simulink model "hopper_3dof_cascade_2"  (R2025a)
settings: Solver=VariableStepAuto  StartTime=0.0  StopTime=36  MaxStep=.005  RelTol=1e-3
values from neighbouring files (symbols this model uses):
  AVI = size_avionics(IN)    [main.m]
  bp = data(:,1)    [load_lookup.m]
  ENGINE = size_engine(IN)    [main.m]
  IN = mission_inputs()    [main.m]
  OUT = Outputs(IN, VEH, TANKS, STRUCT)    [main.m]
  TANKS = size_tanks(IN)    [main.m]
  tbl1 = data(:,2)    [load_lookup.m]
  tbl2 = data(:,3)    [load_lookup.m]
libraries: slpidlib x6, SignalEditorBlockLib x1, cstblocks x1, dspsrcs4 x1
(part 1 of 2)
settings Model: Creator=Espin  LastModifiedBy=asing
settings DebuggingCC: AlgebraicLoopMsg=none

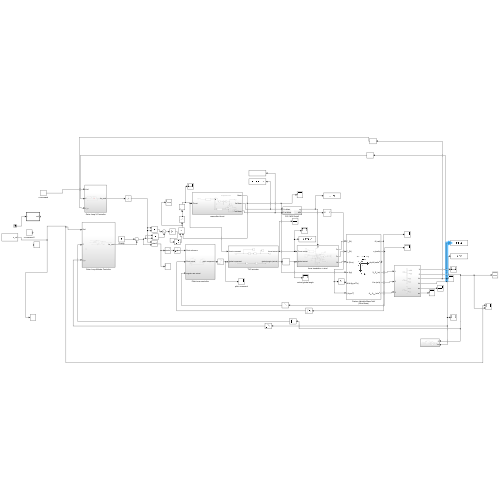
[thumbnail: Simulink's stored preview of the top-level diagram]
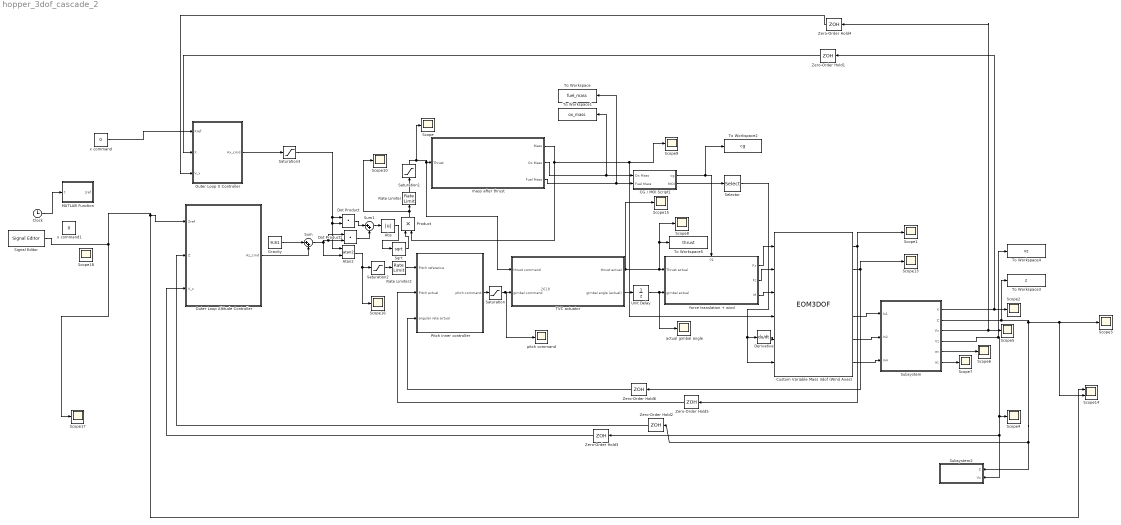
== system hopper_3dof_cascade_2 ==
  note: .2618
  Abs : Abs  SaturateOnIntegerOverflow=off
  Atan2 : Trigonometry  Operator=atan2
  CG / MOI Script1 : Subsystem
  Clock : Clock
  Custom Variable Mass 3dof (Wind Axes) : EOM3DOF  mtype=Custom Variable  v_ini=0
  Derivative : Derivative
  Dot Product : DotProduct  OutDataTypeStr=Inherit: Inherit via internal rule
  Dot Product1 : DotProduct  OutDataTypeStr=Inherit: Inherit via internal rule
  Gravity : Constant  Value=9.81
  MATLAB Function : MATLAB Function  TreatAsAtomicUnit=on
  Outer Loop Altitude Controller : Subsystem
  Outer Loop X Controller : Subsystem
  Pitch inner controller : Subsystem
  Product : Product
  Rate Limiter : RateLimiter  RisingSlewLimit=800  FallingSlewLimit=-800  SampleTimeMode=inherited
  Rate Limiter2 : RateLimiter  RisingSlewLimit=.2618  FallingSlewLimit=-.2618  SampleTimeMode=inherited
  Saturation : Saturate  UpperLimit=.25  LowerLimit=-.25
  Saturation1 : Saturate  UpperLimit=2400  LowerLimit=890  ZeroCross=off
  Saturation2 : Saturate  UpperLimit=.1  LowerLimit=-.1
  Saturation3 : Saturate  UpperLimit=.8  LowerLimit=-.8
  Scope{,1..10,13,15..18} (16 alike) : Scope
      Scope settings: ActiveDisplayYMinimum=624.4996725299402  ActiveDisplayYMaximum=2705.46842252994  DataLoggingVariableName=ScopeData17
      Scope1 settings: ActiveDisplayYMinimum=-0.92499381808462144  ActiveDisplayYMaximum=0.98301480369343519  DataLoggingVariableName=ScopeData4
      Scope10 settings: ActiveDisplayYMinimum=-1  ActiveDisplayYMaximum=1  DataLoggingVariableName=ScopeData18
      Scope13 settings: ActiveDisplayYMinimum=0.23771889209507596  ActiveDisplayYMaximum=0.35709262601864444  DataLoggingVariableName=ScopeData21
      Scope15 settings: ActiveDisplayYMinimum=931.27769507113021  ActiveDisplayYMaximum=1211.8430429766809  DataLoggingVariableName=ScopeData25
      Scope16 settings: ActiveDisplayYMinimum=-0.1222466707090685  ActiveDisplayYMaximum=0.032107185292574392  DataLoggingVariableName=ScopeData26
      Scope17 settings: ActiveDisplayYMinimum=-6.2499999999999982  ActiveDisplayYMaximum=56.25  DataLoggingVariableName=ScopeData31
      Scope18 settings: ActiveDisplayYMinimum=-6.2499999999999982  ActiveDisplayYMaximum=56.25  DataLoggingVariableName=ScopeData39
      Scope2 settings: ActiveDisplayYMinimum=-0.27935542205141428  ActiveDisplayYMaximum=0.36581068662610577  DataLoggingVariableName=ScopeData6
      Scope3 settings: ActiveDisplayYMinimum=-127.57933294479511  ActiveDisplayYMaximum=221.86896869785525  DataLoggingVariableName=ScopeData7
      Scope4 settings: ActiveDisplayYMinimum=-3.5583068913348121  ActiveDisplayYMaximum=0.19242903030250047
      Scope5 settings: ActiveDisplayYMinimum=-962.2230612403514  ActiveDisplayYMaximum=1558.6587762750428  DataLoggingVariableName=ScopeData9
      Scope6 settings: ActiveDisplayYMinimum=-962.2230612403514  ActiveDisplayYMaximum=1558.6587762750428  DataLoggingVariableName=ScopeData10
      Scope7 settings: ActiveDisplayYMinimum=-962.2230612403514  ActiveDisplayYMaximum=1558.6587762750428  DataLoggingVariableName=ScopeData11
      Scope8 settings: ActiveDisplayYMinimum=913.57962331959993  ActiveDisplayYMaximum=1238.5689190055061  DataLoggingVariableName=ScopeData12
      Scope9 settings: ActiveDisplayYMinimum=94.915833260187526  ActiveDisplayYMaximum=94.915892608014829  DataLoggingVariableName=ScopeData13
  Scope14 : Scope  NumInputPorts=2
      settings: ActiveDisplayYMinimum=-3.7499999999999991  ActiveDisplayYMaximum=33.75  DataLoggingVariableName=ScopeData22
  Selector : Selector  NumberOfDimensions=2  InputPortWidth=1  IndexOptions=Index vector (dialog),Index vector (dialog)  Indices=2,2  OutputSizes=1,1
  Signal Editor : SignalEditorBlockLib/Signal Editor  FileName=trajectory2.mat  ActiveScenario=scenario  ActiveSignal=z_ref  IsBus=off  OutputBusObjectStr=Bus: BusObject  SampleTime=0  ZeroCross=off  OutputAfterFinalValue=Setting to zero  Unit=inherit  PreserveSignalName=on  ApplySigPropsToAllScenarios=on  ApplySigPropsToAllSignals=off  SignalPropertySource=Dialog parameters
  Sqrt : Sqrt
  Subsystem : Subsystem
  Subsystem2 : Subsystem
  Sum : Sum  Inputs=|++
  Sum1 : Sum  Inputs=|++
  TVC actuator : Subsystem
  To Workspace : ToWorkspace  VariableName=fuel_mass  SaveFormat=Timeseries  SampleTime=-1
  To Workspace1 : ToWorkspace  VariableName=ox_mass  SaveFormat=Timeseries  SampleTime=-1
  To Workspace2 : ToWorkspace  VariableName=cg  SaveFormat=Timeseries  SampleTime=-1
  To Workspace3 : ToWorkspace  VariableName=z  SaveFormat=Timeseries  SampleTime=-1
  To Workspace4 : ToWorkspace  VariableName=vz  SaveFormat=Timeseries  SampleTime=-1
  To Workspace5 : ToWorkspace  VariableName=thrust  SaveFormat=Timeseries  SampleTime=-1
  Unit Delay : UnitDelay  SampleTime=-1  HasFrameUpgradeWarning=on
  Zero-Order Hold{1..6} (6 alike) : ZeroOrderHold  SampleTime=-1
  actual gimbal angle : Scope
      settings: ActiveDisplayYMinimum=-0.52385024863073193  ActiveDisplayYMaximum=0.68941367272150433  DataLoggingVariableName=ScopeData20
  force translation + wind : Subsystem
      settings: PortSchema="{\"entries\":[{\"content\":{\"sides\":[{\"content\":{\"connectorIds\":[\"In1\",\"In2\"]},\"type\":\"ConnectorPlacement.EquallySpacedRectSide\",\"uuid\":\"479fd6fb-19b9-4dfd-bf6b-42f12e82a54f\"},{\"content\":{\"connectorIds\":[\"Out1\",\"Out2\",\"Out3\"],\"side\":\"RIGHT\"},\"type\":\"ConnectorPlacement.EquallySpacedRectSide\",\"uuid\":\"4df03b8d-1b7e-4664-b5ef-d45791de0677\"},{\"content\":{\"connectorIds\":[\"In3\"],\"side\":\"TOP\"},\"type\":\"ConnectorPlacement.EquallySpacedRectSide\",\"uuid\":\"8e173f4c-8dd7-429b-b7ff-7241e32a3938\"}]},\"type\":\"ConnectorPlacement.EquallySpacedConnector\",\"uuid\":\"4fb4042b-69d2-4473-a071-5f8ab2a018ab\"}],\"packageUris\":[\"http://schema.mathworks.com/mf0/Connector/R2020b\"],\"version\":\"1.0\"}"
  mass after thrust : Subsystem
  pitch command : Scope
      settings: ActiveDisplayYMinimum=-0.18049156336529629  ActiveDisplayYMaximum=0.45484983760747022  DataLoggingVariableName=ScopeData19
  x command : Constant  Value=0
  x command1 : Constant  Value=0
  wires:
  Custom Variable Mass 3dof (Wind Axes)/6 -> Subsystem/3(In4)
  Custom Variable Mass 3dof (Wind Axes)/5 -> Subsystem/2(In2)
  Custom Variable Mass 3dof (Wind Axes)/4 -> Subsystem/1(In1)
  Atan2/1 -> Scope16/1, Saturation2/1
  Pitch inner controller/1(pitch command) -> Saturation/1
  Saturation/1 -> pitch command/1, TVC actuator/2(gimbal command)
  Gravity/1 -> Sum/1
  mass after thrust/1(Mass) -> Product/2, Scope9/1, Custom Variable Mass 3dof (Wind Axes)/4
  Rate Limiter/1 -> Saturation1/1
  Product/1 -> Scope10/1, Rate Limiter/1
  Custom Variable Mass 3dof (Wind Axes)/1 -> Scope1/1, Zero-Order Hold5/1
  Custom Variable Mass 3dof (Wind Axes)/2 -> Scope13/1, Zero-Order Hold6/1
  Subsystem/1(X) -> Zero-Order Hold1/1, Scope2/1
  Subsystem/2(Z) -> To Workspace3/1, Subsystem2/1(Z), Zero-Order Hold2/1, Scope14/2, Scope3/1
  force translation + wind/1(Fx) -> Custom Variable Mass 3dof (Wind Axes)/1
  force translation + wind/3(M) -> Custom Variable Mass 3dof (Wind Axes)/3
  force translation + wind/2(Fz) -> Custom Variable Mass 3dof (Wind Axes)/2
  Subsystem/3(Vx) -> Zero-Order Hold4/1, Scope5/1
  Subsystem/5(ax) -> Scope6/1
  Subsystem/6(az) -> Scope7/1
  Signal Editor/1 -> Scope14/1, Outer Loop Altitude Controller/1(Zref), Scope17/1
  Outer Loop Altitude Controller/1(Az_cmd) -> Sum/2
  Sqrt/1 -> Product/1
  x command/1 -> Outer Loop X Controller/1(Xref)
  Sum/1 -> Dot Product1/1, Dot Product1/2, Atan2/2
  Dot Product/1 -> Sum1/1
  Sum1/1 -> Abs/1
  Dot Product1/1 -> Sum1/2
  Abs/1 -> Sqrt/1
  Outer Loop X Controller/1(Ax_cmd) -> Saturation3/1
  Saturation1/1 -> Scope/1, TVC actuator/1(thrust command), mass after thrust/1(Thrust)
  Zero-Order Hold1/1 -> Outer Loop X Controller/2(X)
  Zero-Order Hold4/1 -> Outer Loop X Controller/3(V_x)
  Zero-Order Hold3/1 -> Outer Loop Altitude Controller/3(V_z)
  Zero-Order Hold2/1 -> Outer Loop Altitude Controller/2(Z)
  Zero-Order Hold5/1 -> Pitch inner controller/2(Pitch actual)
  Zero-Order Hold6/1 -> Pitch inner controller/3(angular rate actual)
  TVC actuator/2(gimbal angle (actual)) -> Unit Delay/1
  Unit Delay/1 -> actual gimbal angle/1, force translation + wind/2(gimbal actual)
  TVC actuator/1(thrust actual) -> Scope8/1, To Workspace5/1, force translation + wind/1(Thrust actual), Scope15/1
  Saturation2/1 -> Rate Limiter2/1
  Rate Limiter2/1 -> Pitch inner controller/1(Pitch reference)
  Saturation3/1 -> Dot Product/1, Atan2/1, Dot Product/2
  mass after thrust/2(Ox Mass) -> To Workspace1/1, CG / MOI Script1/1(Ox Mass)
  mass after thrust/3(Fuel Mass) -> To Workspace/1, CG / MOI Script1/2(Fuel Mass)
  CG / MOI Script1/1(cg) -> To Workspace2/1, force translation + wind/3(cg)
  Derivative/1 -> Custom Variable Mass 3dof (Wind Axes)/5
  CG / MOI Script1/2(MOI) -> Selector/1
  Selector/1 -> Custom Variable Mass 3dof (Wind Axes)/6, Derivative/1
  Clock/1 -> MATLAB Function/1(t)
  Subsystem/4(Vz) -> Subsystem2/2(Vz), Zero-Order Hold3/1, Scope4/1, To Workspace4/1

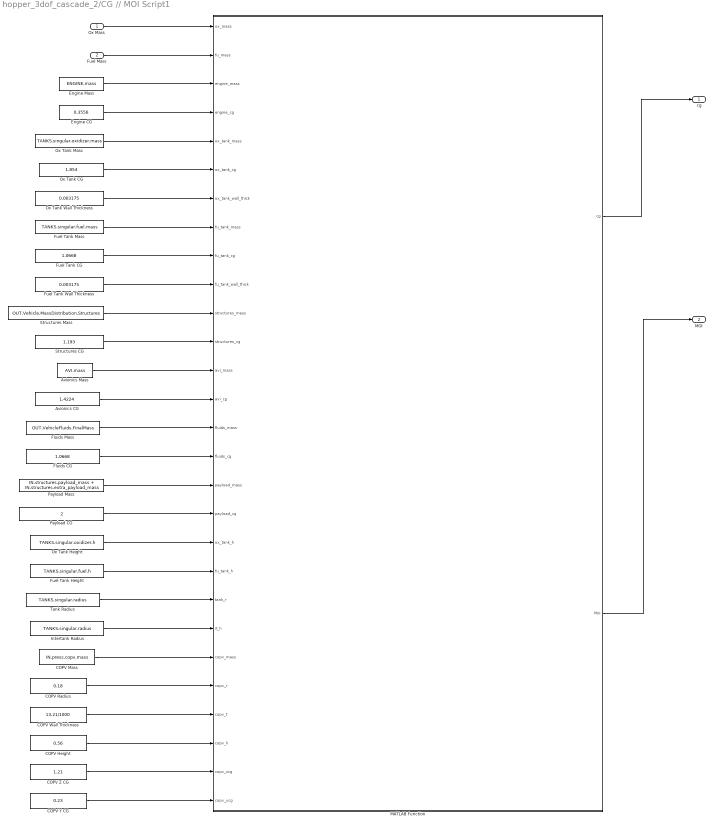
== system hopper_3dof_cascade_2/CG // MOI Script1 ==
  Ox Mass : Inport
  Fuel Mass : Inport  Port=2
  Avionics CG : Constant  Value=1.4224
  Avionics Mass : Constant  Value=AVI.mass
  COPV Height : Constant  Value=0.56
  COPV Mass : Constant  Value=IN.press.copv.mass
  COPV Radius : Constant  Value=0.18
  COPV Wall Thickness : Constant  Value=13.21/1000
  COPV Y CG : Constant  Value=0.23
  COPV Z CG : Constant  Value=1.21
  Engine CG : Constant  Value=0.3556
  Engine Mass : Constant  Value=ENGINE.mass
  Fluids CG : Constant  Value=1.0668
  Fluids Mass : Constant  Value=OUT.VehicleFluids.FinalMass
  Fuel Tank CG : Constant  Value=1.0668
  Fuel Tank Height : Constant  Value=TANKS.singular.fuel.h
  Fuel Tank Mass : Constant  Value=TANKS.singular.fuel.mass
  Fuel Tank Wall Thickness : Constant  Value=0.003175
  Intertank Radius : Constant  Value=TANKS.singular.radius
  MATLAB Function : MATLAB Function  TreatAsAtomicUnit=on
  Ox Tank CG : Constant  Value=1.854
  Ox Tank Height : Constant  Value=TANKS.singular.oxidizer.h
  Ox Tank Mass : Constant  Value=TANKS.singular.oxidizer.mass
  Ox Tank Wall Thickness : Constant  Value=0.003175
  Payload CG : Constant  Value=2
  Payload Mass : Constant  Value=IN.structures.payload_mass + IN.structures.extra_payload_mass
  Structures CG : Constant  Value=1.193
  Structures Mass : Constant  Value=OUT.Vehicle.MassDistribution.Structures
  Tank Radius : Constant  Value=TANKS.singular.radius
  cg : Outport
  MOI : Outport  Port=2
  wires:
  Ox Mass/1 -> MATLAB Function/1(ox_mass)
  Fuel Mass/1 -> MATLAB Function/2(fu_mass)
  Engine Mass/1 -> MATLAB Function/3(engine_mass)
  Engine CG/1 -> MATLAB Function/4(engine_cg)
  Ox Tank Mass/1 -> MATLAB Function/5(ox_tank_mass)
  Ox Tank CG/1 -> MATLAB Function/6(ox_tank_cg)
  Ox Tank Wall Thickness/1 -> MATLAB Function/7(ox_tank_wall_thick)
  Fuel Tank Mass/1 -> MATLAB Function/8(fu_tank_mass)
  Fuel Tank CG/1 -> MATLAB Function/9(fu_tank_cg)
  Fuel Tank Wall Thickness/1 -> MATLAB Function/10(fu_tank_wall_thick)
  Structures Mass/1 -> MATLAB Function/11(structures_mass)
  Structures CG/1 -> MATLAB Function/12(structures_cg)
  Avionics Mass/1 -> MATLAB Function/13(avi_mass)
  Avionics CG/1 -> MATLAB Function/14(avi_cg)
  Fluids Mass/1 -> MATLAB Function/15(fluids_mass)
  Fluids CG/1 -> MATLAB Function/16(fluids_cg)
  Ox Tank Height/1 -> MATLAB Function/19(ox_tank_h)
  Fuel Tank Height/1 -> MATLAB Function/20(fu_tank_h)
  Tank Radius/1 -> MATLAB Function/21(tank_r)
  Intertank Radius/1 -> MATLAB Function/22(it_h)
  MATLAB Function/2(MoI) -> MOI/1
  MATLAB Function/1(cg) -> cg/1
  Payload Mass/1 -> MATLAB Function/17(payload_mass)
  Payload CG/1 -> MATLAB Function/18(payload_cg)
  COPV Mass/1 -> MATLAB Function/23(copv_mass)
  COPV Radius/1 -> MATLAB Function/24(copv_r)
  COPV Height/1 -> MATLAB Function/26(copv_h)
  COPV Z CG/1 -> MATLAB Function/27(copv_zcg)
  COPV Y CG/1 -> MATLAB Function/28(copv_ycg)
  COPV Wall Thickness/1 -> MATLAB Function/25(copv_t)

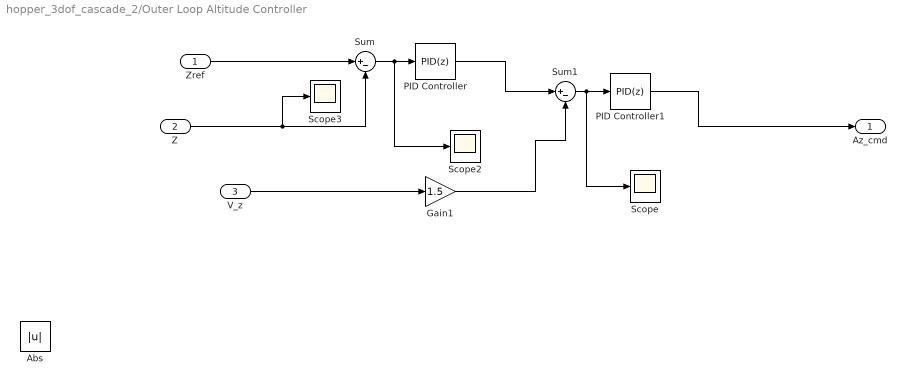
== system hopper_3dof_cascade_2/Outer Loop Altitude Controller ==
  Zref : Inport
  Z : Inport  Port=2
  V_z : Inport  Port=3
  Abs : Abs  SaturateOnIntegerOverflow=off
  Gain1 : Gain  Gain=1.5
  PID Controller : slpidlib/PID Controller  Controller=PID  Form=Parallel  TimeDomain=Discrete-time  UseExternalTs=off  SampleTime=.02  IntegratorMethod=Forward Euler  FilterMethod=Forward Euler  ControllerParametersSource=internal  P=1  I=0  UseKiTs=off  D=0  UseExternalDerivativeSource=off  N=71.8360137365129  UseFilter=off  TunerSelectOption=Transfer Function Based (PID Tuner App)  InitialConditionSource=internal  InitialConditionForIntegrator=0  InitialConditionForFilter=0  DifferentiatorICPrevScaledInput=0  ExternalReset=none  TrackingMode=off  Kt=1  LimitOutput=off  SatLimitsSource=internal  UpperSaturationLimit=inf  LowerSaturationLimit=-inf  LinearizeAsGain=on  AntiWindupMode=none  Kb=1  LimitIntegrator=off  UpperIntegratorSaturationLimit=inf  LowerIntegratorSaturationLimit=-inf  POutMin=[]  POutMax=[]  IOutMin=[]  IOutMax=[]  DOutMin=[]  DOutMax=[]  NOutMin=[]  NOutMax=[]  SumOutMin=[]  SumOutMax=[]  SaturationOutMin=[]  SaturationOutMax=[]  PParamMin=[]  PParamMax=[]  IParamMin=[]  IParamMax=[]  DParamMin=[]  DParamMax=[]  NParamMin=[]  NParamMax=[]  KbParamMin=[]  KbParamMax=[]  KtParamMin=[]  KtParamMax=[]  KbOutMin=[]  KbOutMax=[]  KtOutMin=[]  KtOutMax=[]  IntegratorOutMin=[]  IntegratorOutMax=[]  FilterOutMin=[]  FilterOutMax=[]  SumI1OutMin=[]  SumI1OutMax=[]  SumI2OutMin=[]  SumI2OutMax=[]  SumI3OutMin=[]  SumI3OutMax=[]  SumI4OutMin=[]  SumI4OutMax=[]  SumDOutMin=[]  SumDOutMax=[]  DifferentiatorOutMin=[]  DifferentiatorOutMax=[]  FilterDiffOutCoefMin=[]  FilterDiffOutCoefMax=[]  ReciprocalOutMin=[]  ReciprocalOutMax=[]  SumDenOutMin=[]  SumDenOutMax=[]  SumNumOutMin=[]  SumNumOutMax=[]  DivideOutMin=[]  DivideOutMax=[]  UdiffTsProdOutMin=[]  UdiffTsProdOutMax=[]  NTsProdOutMin=[]  NTsProdOutMax=[]  UintegralTsProdOutMin=[]  UintegralTsProdOutMax=[]  UngainTsProdOutMin=[]  UngainTsProdOutMax=[]  ClampingZeroOutDataTypeStr=Inherit: Inherit via back propagation  ClampingZeroOutMin=[]  ClampingZeroOutMax=[]  FilterDenConstantOutDataTypeStr=Inherit: Inherit via back propagation  FilterDenConstantOutMin=[]  FilterDenConstantOutMax=[]  PCopyOutDataTypeStr=Inherit: Inherit via back propagation  PCopyOutMin=[]  PCopyOutMax=[]  NCopyOutDataTypeStr=Inherit: Inherit via back propagation  NCopyOutMin=[]  NCopyOutMax=[]  IntegratorContinuousStateAttributes=''  IntegratorStateMustResolveToSignalObject=off  IntegratorRTWStateStorageClass=Auto  FilterContinuousStateAttributes=''  FilterStateMustResolveToSignalObject=off  FilterRTWStateStorageClass=Auto  ParallelPVariant=InternalParameters  IdealPVariant=Disabled  IVariant=InternalParameters  DVariant=InternalParameters  IntegratorVariant=Discrete  SatVariant=Disabled  AWVariant=Passthrough  PCopyVariant=Disabled  TRVariant=Disabled  FdbkBlocksVariant=Forward  IdealPFdbkVariant=Disabled  SatFdbkVariant=Disabled  DerivativeFilterVariant=Differentiator  NVariant=Passthrough  NCopyVariant=Disabled_SignalSpec  FilterICVariant=InternalICsDifferentiator  IntegratorICVariant=InternalICs  ExternalResetVariant=Disabled  TRSumVariant=Passthrough  SumFdbkVariant=Disabled  SumVariant=Sum_PID  TsampFilterVariant=InternalTs  TsampNgainVariant=Passthrough  TsampIntegralVariant=Disabled_SignalSpec  ExternalSaturationOutDataTypeStr=Inherit: Same as second input  DerivativeSourceVariant=ErrorSignal  PreIntVariant=InternalPreInt
  PID Controller1 : slpidlib/PID Controller  Controller=PID  Form=Parallel  TimeDomain=Discrete-time  UseExternalTs=off  SampleTime=.02  IntegratorMethod=Forward Euler  FilterMethod=Forward Euler  ControllerParametersSource=internal  P=-5.85683929346037  I=-2.5  UseKiTs=off  D=-0.135933719312933  UseExternalDerivativeSource=off  N=71.8360137365129  UseFilter=off  TunerSelectOption=Transfer Function Based (PID Tuner App)  InitialConditionSource=internal  InitialConditionForIntegrator=0  InitialConditionForFilter=0  DifferentiatorICPrevScaledInput=0  ExternalReset=none  TrackingMode=off  Kt=1  LimitOutput=off  SatLimitsSource=internal  UpperSaturationLimit=inf  LowerSaturationLimit=-inf  LinearizeAsGain=on  AntiWindupMode=none  Kb=1  LimitIntegrator=off  UpperIntegratorSaturationLimit=inf  LowerIntegratorSaturationLimit=-inf  POutMin=[]  POutMax=[]  IOutMin=[]  IOutMax=[]  DOutMin=[]  DOutMax=[]  NOutMin=[]  NOutMax=[]  SumOutMin=[]  SumOutMax=[]  SaturationOutMin=[]  SaturationOutMax=[]  PParamMin=[]  PParamMax=[]  IParamMin=[]  IParamMax=[]  DParamMin=[]  DParamMax=[]  NParamMin=[]  NParamMax=[]  KbParamMin=[]  KbParamMax=[]  KtParamMin=[]  KtParamMax=[]  KbOutMin=[]  KbOutMax=[]  KtOutMin=[]  KtOutMax=[]  IntegratorOutMin=[]  IntegratorOutMax=[]  FilterOutMin=[]  FilterOutMax=[]  SumI1OutMin=[]  SumI1OutMax=[]  SumI2OutMin=[]  SumI2OutMax=[]  SumI3OutMin=[]  SumI3OutMax=[]  SumI4OutMin=[]  SumI4OutMax=[]  SumDOutMin=[]  SumDOutMax=[]  DifferentiatorOutMin=[]  DifferentiatorOutMax=[]  FilterDiffOutCoefMin=[]  FilterDiffOutCoefMax=[]  ReciprocalOutMin=[]  ReciprocalOutMax=[]  SumDenOutMin=[]  SumDenOutMax=[]  SumNumOutMin=[]  SumNumOutMax=[]  DivideOutMin=[]  DivideOutMax=[]  UdiffTsProdOutMin=[]  UdiffTsProdOutMax=[]  NTsProdOutMin=[]  NTsProdOutMax=[]  UintegralTsProdOutMin=[]  UintegralTsProdOutMax=[]  UngainTsProdOutMin=[]  UngainTsProdOutMax=[]  ClampingZeroOutDataTypeStr=Inherit: Inherit via back propagation  ClampingZeroOutMin=[]  ClampingZeroOutMax=[]  FilterDenConstantOutDataTypeStr=Inherit: Inherit via back propagation  FilterDenConstantOutMin=[]  FilterDenConstantOutMax=[]  PCopyOutDataTypeStr=Inherit: Inherit via back propagation  PCopyOutMin=[]  PCopyOutMax=[]  NCopyOutDataTypeStr=Inherit: Inherit via back propagation  NCopyOutMin=[]  NCopyOutMax=[]  IntegratorContinuousStateAttributes=''  IntegratorStateMustResolveToSignalObject=off  IntegratorRTWStateStorageClass=Auto  FilterContinuousStateAttributes=''  FilterStateMustResolveToSignalObject=off  FilterRTWStateStorageClass=Auto  ParallelPVariant=InternalParameters  IdealPVariant=Disabled  IVariant=InternalParameters  DVariant=InternalParameters  IntegratorVariant=Discrete  SatVariant=Disabled  AWVariant=Passthrough  PCopyVariant=Disabled  TRVariant=Disabled  FdbkBlocksVariant=Forward  IdealPFdbkVariant=Disabled  SatFdbkVariant=Disabled  DerivativeFilterVariant=Differentiator  NVariant=Passthrough  NCopyVariant=Disabled_SignalSpec  FilterICVariant=InternalICsDifferentiator  IntegratorICVariant=InternalICs  ExternalResetVariant=Disabled  TRSumVariant=Passthrough  SumFdbkVariant=Disabled  SumVariant=Sum_PID  TsampFilterVariant=InternalTs  TsampNgainVariant=Passthrough  TsampIntegralVariant=Disabled_SignalSpec  ExternalSaturationOutDataTypeStr=Inherit: Same as second input  DerivativeSourceVariant=ErrorSignal  PreIntVariant=InternalPreInt
  Scope : Scope
      settings: ActiveDisplayYMinimum=-2431.2435931386744  ActiveDisplayYMaximum=870.07655995958  DataLoggingVariableName=ScopeData27
  Scope2 : Scope
      settings: ActiveDisplayYMinimum=-1450.1308335174933  ActiveDisplayYMaximum=480.08268664272219  DataLoggingVariableName=ScopeData29
  Scope3 : Scope
      settings: ActiveDisplayYMinimum=-2628.2294879970932  ActiveDisplayYMaximum=1011.4759807937319  DataLoggingVariableName=ScopeData30
  Sum : Sum  Inputs=|+-
  Sum1 : Sum  Inputs=|+-
  Az_cmd : Outport
  wires:
  Zref/1 -> Sum/1
  PID Controller1/1 -> Az_cmd/1
  Sum/1 -> Scope2/1, PID Controller/1
  V_z/1 -> Gain1/1
  Sum1/1 -> Scope/1, PID Controller1/1
  Z/1 -> Scope3/1, Sum/2
  PID Controller/1 -> Sum1/1
  Gain1/1 -> Sum1/2

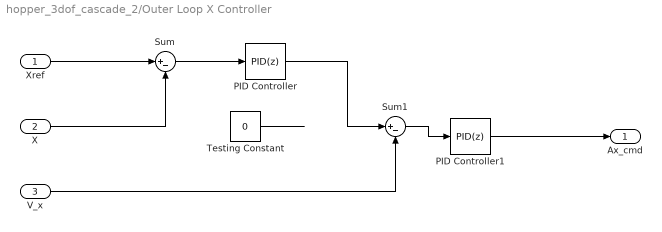
== system hopper_3dof_cascade_2/Outer Loop X Controller ==
  Xref : Inport
  X : Inport  Port=2
  V_x : Inport  Port=3
  PID Controller : slpidlib/PID Controller  Controller=PID  Form=Parallel  TimeDomain=Discrete-time  UseExternalTs=off  SampleTime=0.02  IntegratorMethod=Forward Euler  FilterMethod=Forward Euler  ControllerParametersSource=internal  P=1.29719139291204  I=0.0566995131971568  UseKiTs=off  D=2.20404079588237  UseExternalDerivativeSource=off  N=69.2081994586311  UseFilter=on  TunerSelectOption=Transfer Function Based (PID Tuner App)  InitialConditionSource=internal  InitialConditionForIntegrator=0  InitialConditionForFilter=0  DifferentiatorICPrevScaledInput=0  ExternalReset=none  TrackingMode=off  Kt=1  LimitOutput=off  SatLimitsSource=internal  UpperSaturationLimit=inf  LowerSaturationLimit=-inf  LinearizeAsGain=on  AntiWindupMode=none  Kb=1  LimitIntegrator=off  UpperIntegratorSaturationLimit=inf  LowerIntegratorSaturationLimit=-inf  POutMin=[]  POutMax=[]  IOutMin=[]  IOutMax=[]  DOutMin=[]  DOutMax=[]  NOutMin=[]  NOutMax=[]  SumOutMin=[]  SumOutMax=[]  SaturationOutMin=[]  SaturationOutMax=[]  PParamMin=[]  PParamMax=[]  IParamMin=[]  IParamMax=[]  DParamMin=[]  DParamMax=[]  NParamMin=[]  NParamMax=[]  KbParamMin=[]  KbParamMax=[]  KtParamMin=[]  KtParamMax=[]  KbOutMin=[]  KbOutMax=[]  KtOutMin=[]  KtOutMax=[]  IntegratorOutMin=[]  IntegratorOutMax=[]  FilterOutMin=[]  FilterOutMax=[]  SumI1OutMin=[]  SumI1OutMax=[]  SumI2OutMin=[]  SumI2OutMax=[]  SumI3OutMin=[]  SumI3OutMax=[]  SumI4OutMin=[]  SumI4OutMax=[]  SumDOutMin=[]  SumDOutMax=[]  DifferentiatorOutMin=[]  DifferentiatorOutMax=[]  FilterDiffOutCoefMin=[]  FilterDiffOutCoefMax=[]  ReciprocalOutMin=[]  ReciprocalOutMax=[]  SumDenOutMin=[]  SumDenOutMax=[]  SumNumOutMin=[]  SumNumOutMax=[]  DivideOutMin=[]  DivideOutMax=[]  UdiffTsProdOutMin=[]  UdiffTsProdOutMax=[]  NTsProdOutMin=[]  NTsProdOutMax=[]  UintegralTsProdOutMin=[]  UintegralTsProdOutMax=[]  UngainTsProdOutMin=[]  UngainTsProdOutMax=[]  ClampingZeroOutDataTypeStr=Inherit: Inherit via back propagation  ClampingZeroOutMin=[]  ClampingZeroOutMax=[]  FilterDenConstantOutDataTypeStr=Inherit: Inherit via back propagation  FilterDenConstantOutMin=[]  FilterDenConstantOutMax=[]  PCopyOutDataTypeStr=Inherit: Inherit via back propagation  PCopyOutMin=[]  PCopyOutMax=[]  NCopyOutDataTypeStr=Inherit: Inherit via back propagation  NCopyOutMin=[]  NCopyOutMax=[]  IntegratorContinuousStateAttributes=''  IntegratorStateMustResolveToSignalObject=off  IntegratorRTWStateStorageClass=Auto  FilterContinuousStateAttributes=''  FilterStateMustResolveToSignalObject=off  FilterRTWStateStorageClass=Auto  ParallelPVariant=InternalParameters  IdealPVariant=Disabled  IVariant=InternalParameters  DVariant=InternalParameters  IntegratorVariant=Discrete  SatVariant=Disabled  AWVariant=Passthrough  PCopyVariant=Disabled  TRVariant=Disabled  FdbkBlocksVariant=Forward  IdealPFdbkVariant=Disabled  SatFdbkVariant=Disabled  DerivativeFilterVariant=ForwardEulerFilter  NVariant=InternalParameters  NCopyVariant=Disabled  FilterICVariant=InternalICsFilter  IntegratorICVariant=InternalICs  ExternalResetVariant=Disabled  TRSumVariant=Passthrough  SumFdbkVariant=Disabled  SumVariant=Sum_PID  TsampFilterVariant=InternalTs  TsampNgainVariant=Passthrough  TsampIntegralVariant=Disabled_SignalSpec  ExternalSaturationOutDataTypeStr=Inherit: Same as second input  DerivativeSourceVariant=ErrorSignal  PreIntVariant=InternalPreInt
  PID Controller1 : slpidlib/PID Controller  Controller=PID  Form=Parallel  TimeDomain=Discrete-time  UseExternalTs=off  SampleTime=0.02  IntegratorMethod=Forward Euler  FilterMethod=Forward Euler  ControllerParametersSource=internal  P=-0.620873856451215  I=-0.0720838118169977  UseKiTs=off  D=0.0949165148503063  UseExternalDerivativeSource=off  N=6.13296091836775  UseFilter=on  TunerSelectOption=Transfer Function Based (PID Tuner App)  InitialConditionSource=internal  InitialConditionForIntegrator=0  InitialConditionForFilter=0  DifferentiatorICPrevScaledInput=0  ExternalReset=none  TrackingMode=off  Kt=1  LimitOutput=off  SatLimitsSource=internal  UpperSaturationLimit=inf  LowerSaturationLimit=-inf  LinearizeAsGain=on  AntiWindupMode=none  Kb=1  LimitIntegrator=off  UpperIntegratorSaturationLimit=inf  LowerIntegratorSaturationLimit=-inf  POutMin=[]  POutMax=[]  IOutMin=[]  IOutMax=[]  DOutMin=[]  DOutMax=[]  NOutMin=[]  NOutMax=[]  SumOutMin=[]  SumOutMax=[]  SaturationOutMin=[]  SaturationOutMax=[]  PParamMin=[]  PParamMax=[]  IParamMin=[]  IParamMax=[]  DParamMin=[]  DParamMax=[]  NParamMin=[]  NParamMax=[]  KbParamMin=[]  KbParamMax=[]  KtParamMin=[]  KtParamMax=[]  KbOutMin=[]  KbOutMax=[]  KtOutMin=[]  KtOutMax=[]  IntegratorOutMin=[]  IntegratorOutMax=[]  FilterOutMin=[]  FilterOutMax=[]  SumI1OutMin=[]  SumI1OutMax=[]  SumI2OutMin=[]  SumI2OutMax=[]  SumI3OutMin=[]  SumI3OutMax=[]  SumI4OutMin=[]  SumI4OutMax=[]  SumDOutMin=[]  SumDOutMax=[]  DifferentiatorOutMin=[]  DifferentiatorOutMax=[]  FilterDiffOutCoefMin=[]  FilterDiffOutCoefMax=[]  ReciprocalOutMin=[]  ReciprocalOutMax=[]  SumDenOutMin=[]  SumDenOutMax=[]  SumNumOutMin=[]  SumNumOutMax=[]  DivideOutMin=[]  DivideOutMax=[]  UdiffTsProdOutMin=[]  UdiffTsProdOutMax=[]  NTsProdOutMin=[]  NTsProdOutMax=[]  UintegralTsProdOutMin=[]  UintegralTsProdOutMax=[]  UngainTsProdOutMin=[]  UngainTsProdOutMax=[]  ClampingZeroOutDataTypeStr=Inherit: Inherit via back propagation  ClampingZeroOutMin=[]  ClampingZeroOutMax=[]  FilterDenConstantOutDataTypeStr=Inherit: Inherit via back propagation  FilterDenConstantOutMin=[]  FilterDenConstantOutMax=[]  PCopyOutDataTypeStr=Inherit: Inherit via back propagation  PCopyOutMin=[]  PCopyOutMax=[]  NCopyOutDataTypeStr=Inherit: Inherit via back propagation  NCopyOutMin=[]  NCopyOutMax=[]  IntegratorContinuousStateAttributes=''  IntegratorStateMustResolveToSignalObject=off  IntegratorRTWStateStorageClass=Auto  FilterContinuousStateAttributes=''  FilterStateMustResolveToSignalObject=off  FilterRTWStateStorageClass=Auto  ParallelPVariant=InternalParameters  IdealPVariant=Disabled  IVariant=InternalParameters  DVariant=InternalParameters  IntegratorVariant=Discrete  SatVariant=Disabled  AWVariant=Passthrough  PCopyVariant=Disabled  TRVariant=Disabled  FdbkBlocksVariant=Forward  IdealPFdbkVariant=Disabled  SatFdbkVariant=Disabled  DerivativeFilterVariant=ForwardEulerFilter  NVariant=InternalParameters  NCopyVariant=Disabled  FilterICVariant=InternalICsFilter  IntegratorICVariant=InternalICs  ExternalResetVariant=Disabled  TRSumVariant=Passthrough  SumFdbkVariant=Disabled  SumVariant=Sum_PID  TsampFilterVariant=InternalTs  TsampNgainVariant=Passthrough  TsampIntegralVariant=Disabled_SignalSpec  ExternalSaturationOutDataTypeStr=Inherit: Same as second input  DerivativeSourceVariant=ErrorSignal  PreIntVariant=InternalPreInt
  Sum : Sum  Inputs=|+-
  Sum1 : Sum  Inputs=|+-
  Testing Constant : Constant  Value=0
  Ax_cmd : Outport
  wires:
  Xref/1 -> Sum/1
  PID Controller1/1 -> Ax_cmd/1
  Sum/1 -> PID Controller/1
  X/1 -> Sum/2
  PID Controller/1 -> Sum1/1
  V_x/1 -> Sum1/2
  Testing Constant/1 -> ?
  Sum1/1 -> PID Controller1/1

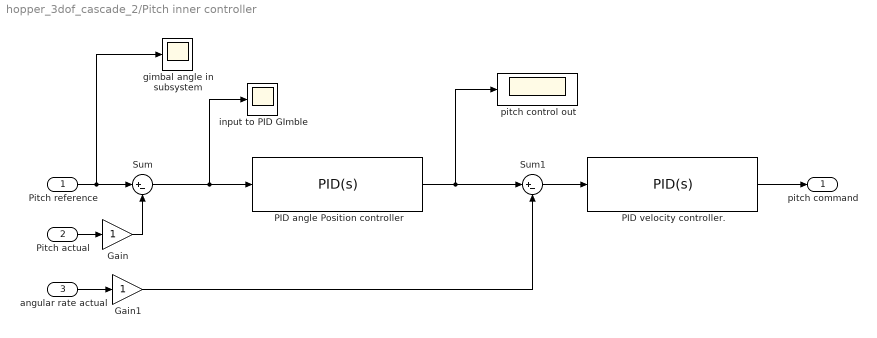
== system hopper_3dof_cascade_2/Pitch inner controller ==
  Pitch reference : Inport
  Pitch actual : Inport  Port=2
  angular rate actual : Inport  Port=3
  Gain : Gain
  Gain1 : Gain
  PID angle Position controller : slpidlib/PID Controller  Controller=PID  Form=Parallel  TimeDomain=Continuous-time  UseExternalTs=off  SampleTime=.01  IntegratorMethod=Forward Euler  FilterMethod=Forward Euler  ControllerParametersSource=internal  P=2.71925952557616  I=0.432929489163779  UseKiTs=off  D=0.921646829283693  UseExternalDerivativeSource=off  N=202.456655722126  UseFilter=on  TunerSelectOption=Transfer Function Based (PID Tuner App)  InitialConditionSource=internal  InitialConditionForIntegrator=0  InitialConditionForFilter=0  DifferentiatorICPrevScaledInput=0  ExternalReset=none  TrackingMode=off  Kt=1  LimitOutput=off  SatLimitsSource=internal  UpperSaturationLimit=inf  LowerSaturationLimit=-inf  LinearizeAsGain=on  AntiWindupMode=none  Kb=1  LimitIntegrator=off  UpperIntegratorSaturationLimit=inf  LowerIntegratorSaturationLimit=-inf  POutMin=[]  POutMax=[]  IOutMin=[]  IOutMax=[]  DOutMin=[]  DOutMax=[]  NOutMin=[]  NOutMax=[]  SumOutMin=[]  SumOutMax=[]  SaturationOutMin=[]  SaturationOutMax=[]  PParamMin=[]  PParamMax=[]  IParamMin=[]  IParamMax=[]  DParamMin=[]  DParamMax=[]  NParamMin=[]  NParamMax=[]  KbParamMin=[]  KbParamMax=[]  KtParamMin=[]  KtParamMax=[]  KbOutMin=[]  KbOutMax=[]  KtOutMin=[]  KtOutMax=[]  IntegratorOutMin=[]  IntegratorOutMax=[]  FilterOutMin=[]  FilterOutMax=[]  SumI1OutMin=[]  SumI1OutMax=[]  SumI2OutMin=[]  SumI2OutMax=[]  SumI3OutMin=[]  SumI3OutMax=[]  SumI4OutMin=[]  SumI4OutMax=[]  SumDOutMin=[]  SumDOutMax=[]  DifferentiatorOutMin=[]  DifferentiatorOutMax=[]  FilterDiffOutCoefMin=[]  FilterDiffOutCoefMax=[]  ReciprocalOutMin=[]  ReciprocalOutMax=[]  SumDenOutMin=[]  SumDenOutMax=[]  SumNumOutMin=[]  SumNumOutMax=[]  DivideOutMin=[]  DivideOutMax=[]  UdiffTsProdOutMin=[]  UdiffTsProdOutMax=[]  NTsProdOutMin=[]  NTsProdOutMax=[]  UintegralTsProdOutMin=[]  UintegralTsProdOutMax=[]  UngainTsProdOutMin=[]  UngainTsProdOutMax=[]  ClampingZeroOutDataTypeStr=Inherit: Inherit via back propagation  ClampingZeroOutMin=[]  ClampingZeroOutMax=[]  FilterDenConstantOutDataTypeStr=Inherit: Inherit via back propagation  FilterDenConstantOutMin=[]  FilterDenConstantOutMax=[]  PCopyOutDataTypeStr=Inherit: Inherit via back propagation  PCopyOutMin=[]  PCopyOutMax=[]  NCopyOutDataTypeStr=Inherit: Inherit via back propagation  NCopyOutMin=[]  NCopyOutMax=[]  IntegratorContinuousStateAttributes=''  IntegratorStateMustResolveToSignalObject=off  IntegratorRTWStateStorageClass=Auto  FilterContinuousStateAttributes=''  FilterStateMustResolveToSignalObject=off  FilterRTWStateStorageClass=Auto  ParallelPVariant=InternalParameters  IdealPVariant=Disabled  IVariant=InternalParameters  DVariant=InternalParameters  IntegratorVariant=Continuous  SatVariant=Disabled  AWVariant=Passthrough  PCopyVariant=Disabled  TRVariant=Disabled  FdbkBlocksVariant=Forward  IdealPFdbkVariant=Disabled  SatFdbkVariant=Disabled  DerivativeFilterVariant=ContFilter  NVariant=InternalParameters  NCopyVariant=Disabled  FilterICVariant=InternalICsFilter  IntegratorICVariant=InternalICs  ExternalResetVariant=Disabled  TRSumVariant=Passthrough  SumFdbkVariant=Disabled  SumVariant=Sum_PID  TsampFilterVariant=InternalTs  TsampNgainVariant=Passthrough  TsampIntegralVariant=Disabled_SignalSpec  ExternalSaturationOutDataTypeStr=Inherit: Same as second input  DerivativeSourceVariant=ErrorSignal  PreIntVariant=InternalPreInt
  PID velocity controller. : slpidlib/PID Controller  Controller=PID  Form=Parallel  TimeDomain=Continuous-time  UseExternalTs=off  SampleTime=.01  IntegratorMethod=Forward Euler  FilterMethod=Forward Euler  ControllerParametersSource=internal  P=0.0125882721746036  I=0.00136230972396466  UseKiTs=off  D=0.023343460151588  UseExternalDerivativeSource=off  N=1.99025149076839  UseFilter=on  TunerSelectOption=Transfer Function Based (PID Tuner App)  InitialConditionSource=internal  InitialConditionForIntegrator=0  InitialConditionForFilter=0  DifferentiatorICPrevScaledInput=0  ExternalReset=none  TrackingMode=off  Kt=1  LimitOutput=off  SatLimitsSource=internal  UpperSaturationLimit=inf  LowerSaturationLimit=-inf  LinearizeAsGain=on  AntiWindupMode=none  Kb=1  LimitIntegrator=off  UpperIntegratorSaturationLimit=inf  LowerIntegratorSaturationLimit=-inf  POutMin=[]  POutMax=[]  IOutMin=[]  IOutMax=[]  DOutMin=[]  DOutMax=[]  NOutMin=[]  NOutMax=[]  SumOutMin=[]  SumOutMax=[]  SaturationOutMin=[]  SaturationOutMax=[]  PParamMin=[]  PParamMax=[]  IParamMin=[]  IParamMax=[]  DParamMin=[]  DParamMax=[]  NParamMin=[]  NParamMax=[]  KbParamMin=[]  KbParamMax=[]  KtParamMin=[]  KtParamMax=[]  KbOutMin=[]  KbOutMax=[]  KtOutMin=[]  KtOutMax=[]  IntegratorOutMin=[]  IntegratorOutMax=[]  FilterOutMin=[]  FilterOutMax=[]  SumI1OutMin=[]  SumI1OutMax=[]  SumI2OutMin=[]  SumI2OutMax=[]  SumI3OutMin=[]  SumI3OutMax=[]  SumI4OutMin=[]  SumI4OutMax=[]  SumDOutMin=[]  SumDOutMax=[]  DifferentiatorOutMin=[]  DifferentiatorOutMax=[]  FilterDiffOutCoefMin=[]  FilterDiffOutCoefMax=[]  ReciprocalOutMin=[]  ReciprocalOutMax=[]  SumDenOutMin=[]  SumDenOutMax=[]  SumNumOutMin=[]  SumNumOutMax=[]  DivideOutMin=[]  DivideOutMax=[]  UdiffTsProdOutMin=[]  UdiffTsProdOutMax=[]  NTsProdOutMin=[]  NTsProdOutMax=[]  UintegralTsProdOutMin=[]  UintegralTsProdOutMax=[]  UngainTsProdOutMin=[]  UngainTsProdOutMax=[]  ClampingZeroOutDataTypeStr=Inherit: Inherit via back propagation  ClampingZeroOutMin=[]  ClampingZeroOutMax=[]  FilterDenConstantOutDataTypeStr=Inherit: Inherit via back propagation  FilterDenConstantOutMin=[]  FilterDenConstantOutMax=[]  PCopyOutDataTypeStr=Inherit: Inherit via back propagation  PCopyOutMin=[]  PCopyOutMax=[]  NCopyOutDataTypeStr=Inherit: Inherit via back propagation  NCopyOutMin=[]  NCopyOutMax=[]  IntegratorContinuousStateAttributes=''  IntegratorStateMustResolveToSignalObject=off  IntegratorRTWStateStorageClass=Auto  FilterContinuousStateAttributes=''  FilterStateMustResolveToSignalObject=off  FilterRTWStateStorageClass=Auto  ParallelPVariant=InternalParameters  IdealPVariant=Disabled  IVariant=InternalParameters  DVariant=InternalParameters  IntegratorVariant=Continuous  SatVariant=Disabled  AWVariant=Passthrough  PCopyVariant=Disabled  TRVariant=Disabled  FdbkBlocksVariant=Forward  IdealPFdbkVariant=Disabled  SatFdbkVariant=Disabled  DerivativeFilterVariant=ContFilter  NVariant=InternalParameters  NCopyVariant=Disabled  FilterICVariant=InternalICsFilter  IntegratorICVariant=InternalICs  ExternalResetVariant=Disabled  TRSumVariant=Passthrough  SumFdbkVariant=Disabled  SumVariant=Sum_PID  TsampFilterVariant=InternalTs  TsampNgainVariant=Passthrough  TsampIntegralVariant=Disabled_SignalSpec  ExternalSaturationOutDataTypeStr=Inherit: Same as second input  DerivativeSourceVariant=ErrorSignal  PreIntVariant=InternalPreInt
  Sum : Sum  Inputs=|+-
  Sum1 : Sum  Inputs=|+-
  gimbal angle in subsystem : Scope
      settings: ActiveDisplayYMinimum=-0.050908038627042115  ActiveDisplayYMaximum=0.037591083917641  DataLoggingVariableName=ScopeData34
  input to PID GImble : Scope
      settings: ActiveDisplayYMinimum=-4.3031232761314806  ActiveDisplayYMaximum=2.5199807787902841  DataLoggingVariableName=ScopeData32
  pitch control out : Scope
      settings: ActiveDisplayYMinimum=6.4844722385980127E-5  ActiveDisplayYMaximum=0.015867649870164591  DataLoggingVariableName=ScopeData33
  pitch command : Outport
  wires:
  Pitch reference/1 -> gimbal angle in subsystem/1, Sum/1
  Pitch actual/1 -> Gain/1
  Gain/1 -> Sum/2
  Sum/1 -> input to PID GImble/1, PID angle Position controller/1
  PID angle Position controller/1 -> Sum1/1, pitch control out/1
  angular rate actual/1 -> Gain1/1
  Gain1/1 -> Sum1/2
  Sum1/1 -> PID velocity controller./1
  PID velocity controller./1 -> pitch command/1

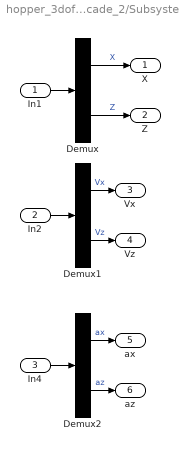
== system hopper_3dof_cascade_2/Subsystem ==
  In1 : Inport
  In2 : Inport  Port=2
  In4 : Inport  Port=3
  Demux : Demux  Outputs=2
  Demux1 : Demux  Outputs=2
  Demux2 : Demux  Outputs=2
  X : Outport
  Z : Outport  Port=2
  Vx : Outport  Port=3
  Vz : Outport  Port=4
  ax : Outport  Port=5
  az : Outport  Port=6
  wires:
  Demux1/2 -> Vz/1  "Vz"
  In2/1 -> Demux1/1
  Demux1/1 -> Vx/1  "Vx"
  In1/1 -> Demux/1
  Demux/2 -> Z/1  "Z"
  Demux/1 -> X/1  "X"
  Demux2/1 -> ax/1  "ax"
  Demux2/2 -> az/1  "az"
  In4/1 -> Demux2/1

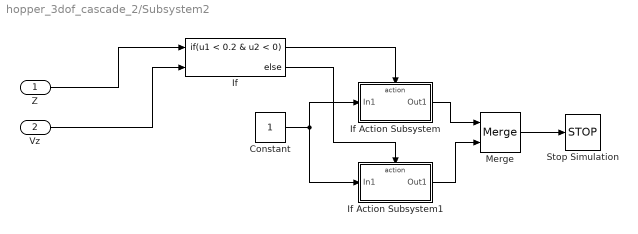
== system hopper_3dof_cascade_2/Subsystem2 ==
  Z : Inport
  Vz : Inport  Port=2
  Constant : Constant
  If : If  NumInputs=2  IfExpression=u1 < 0.2 & u2 < 0
  If Action Subsystem : Subsystem  TreatAsAtomicUnit=on
  If Action Subsystem1 : Subsystem  TreatAsAtomicUnit=on
  Merge : Merge
  Stop Simulation : Stop
  wires:
  Z/1 -> If/1
  Vz/1 -> If/2
  If/1 -> If Action Subsystem/Action
  If/2 -> If Action Subsystem1/Action
  Constant/1 -> If Action Subsystem1/1(In1), If Action Subsystem/1(In1)
  If Action Subsystem/1(Out1) -> Merge/1
  If Action Subsystem1/1(Out1) -> Merge/2
  Merge/1 -> Stop Simulation/1

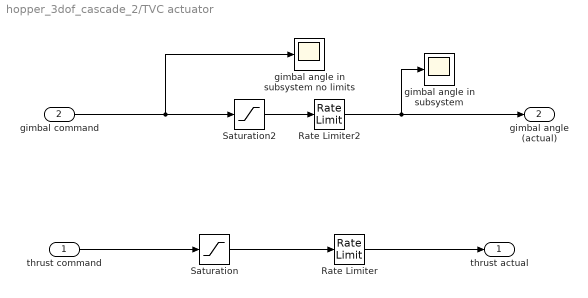
== system hopper_3dof_cascade_2/TVC actuator ==
  thrust command : Inport
  gimbal command : Inport  Port=2
  Rate Limiter : RateLimiter  RisingSlewLimit=800  FallingSlewLimit=-800  SampleTimeMode=inherited
  Rate Limiter2 : RateLimiter  RisingSlewLimit=.2618  FallingSlewLimit=-.2618  SampleTimeMode=inherited
  Saturation : Saturate  UpperLimit=2400  LowerLimit=890
  Saturation2 : Saturate  UpperLimit=.2618  LowerLimit=-.2618
  gimbal angle in subsystem : Scope
      settings: ActiveDisplayYMinimum=-0.027763262466734467  ActiveDisplayYMaximum=0.0055911260638454568
  gimbal angle in subsystem no limits : Scope
      settings: ActiveDisplayYMinimum=-0.050908038627042115  ActiveDisplayYMaximum=0.037591083917641  DataLoggingVariableName=ScopeData28
  thrust actual : Outport
  gimbal angle (actual) : Outport  Port=2
  wires:
  gimbal command/1 -> gimbal angle in subsystem no limits/1, Saturation2/1
  Saturation2/1 -> Rate Limiter2/1
  Rate Limiter2/1 -> gimbal angle (actual)/1, gimbal angle in subsystem/1
  Saturation/1 -> Rate Limiter/1
  thrust command/1 -> Saturation/1
  Rate Limiter/1 -> thrust actual/1

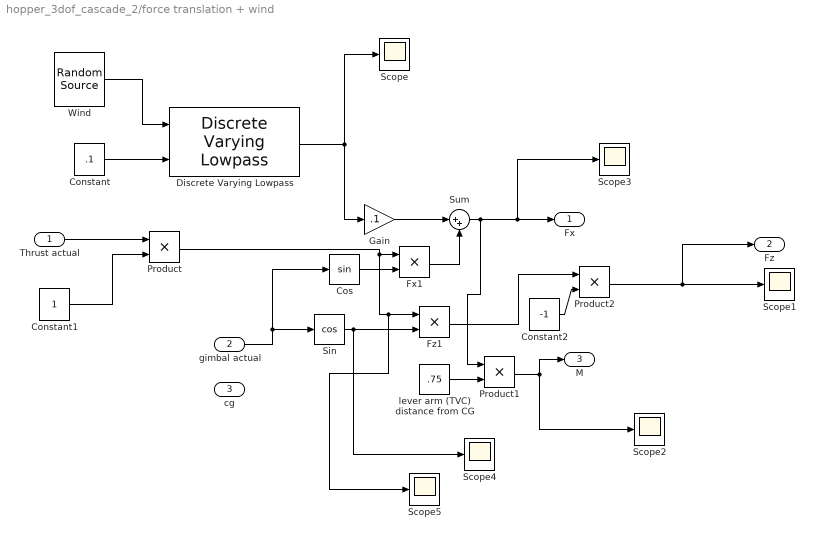
== system hopper_3dof_cascade_2/force translation + wind ==
  Thrust actual : Inport
  gimbal actual : Inport  Port=2
  cg : Inport  Port=3
  Constant : Constant  Value=.1
  Constant1 : Constant
  Constant2 : Constant  Value=-1
  Cos : Trigonometry
  Discrete Varying Lowpass : cstblocks/Linear Parameter Varying/Discrete Varying Lowpass  N=2  w0=0  Ts=1
  Fx1 : Product
  Fz1 : Product
  Gain : Gain  Gain=.1
  Product : Product
  Product1 : Product
  Product2 : Product
  Scope{,1..5} (6 alike) : Scope
      Scope settings: ActiveDisplayYMinimum=-7.9183590464792282  ActiveDisplayYMaximum=51.900530683426176  DataLoggingVariableName=ScopeData8
      Scope1 settings: ActiveDisplayYMinimum=-1  ActiveDisplayYMaximum=1  DataLoggingVariableName=ScopeData14
      Scope2 settings: ActiveDisplayYMinimum=-1  ActiveDisplayYMaximum=1  DataLoggingVariableName=ScopeData15
      Scope3 settings: ActiveDisplayYMinimum=-1  ActiveDisplayYMaximum=1  DataLoggingVariableName=ScopeData16
      Scope4 settings: ActiveDisplayYMinimum=0.96584493866804921  ActiveDisplayYMaximum=0.99170987981187175  DataLoggingVariableName=ScopeData23
      Scope5 settings: ActiveDisplayYMinimum=837.04346660798183  ActiveDisplayYMaximum=1638.9745482042581  DataLoggingVariableName=ScopeData24
  Sin : Trigonometry  Operator=cos
  Sum : Sum  Inputs=|++
  Wind : dspsrcs4/Random Source  SrcType=Gaussian  MinVal=0  MaxVal=1  MeanVal=50  VarVal=1000  RepMode=Specify seed  rawSeed=1  IsInherit=off  SampTime=0.2  SampFrame=1  OutComplex=Real  DataType=double  SimulateUsing=Interpreted execution
  lever arm (TVC) distance from CG : Constant  Value=.75
  Fx : Outport
  Fz : Outport  Port=2
  M : Outport  Port=3
  wires:
  Constant/1 -> Discrete Varying Lowpass/2
  Discrete Varying Lowpass/1 -> Gain/1, Scope/1
  Wind/1 -> Discrete Varying Lowpass/1
  Sum/1 -> Product1/1, Scope3/1, Fx/1
  gimbal actual/1 -> Cos/1, Sin/1
  Product1/1 -> Scope2/1, M/1
  Fx1/1 -> Sum/2
  Sin/1 -> Scope4/1, Fz1/2
  Cos/1 -> Fx1/2
  lever arm (TVC) distance from CG/1 -> Product1/2
  Product/1 -> Scope5/1, Fz1/1, Fx1/1
  Thrust actual/1 -> Product/1
  Constant1/1 -> Product/2
  Fz1/1 -> Product2/1
  Constant2/1 -> Product2/2
  Product2/1 -> Fz/1, Scope1/1
  Gain/1 -> Sum/1

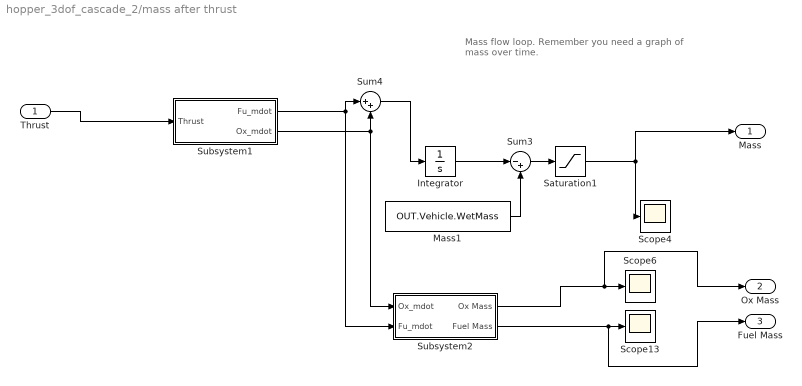
== system hopper_3dof_cascade_2/mass after thrust ==
  note: Mass flow loop. Remember you need a graph of mass over time.
  Thrust : Inport
  Integrator : Integrator
  Mass1 : Constant  Value=OUT.Vehicle.WetMass
  Saturation1 : Saturate  UpperLimit=OUT.Vehicle.WetMass  LowerLimit=OUT.Vehicle.DryMass
  Scope13 : Scope
      settings: ActiveDisplayYMinimum=3.7124260392916559  ActiveDisplayYMaximum=9.5875082178564828  DataLoggingVariableName=ScopeData2
  Scope4 : Scope
      settings: ActiveDisplayYMinimum=87.779536141867183  ActiveDisplayYMaximum=112.03927836942441  DataLoggingVariableName=ScopeData3
  Scope6 : Scope
      settings: ActiveDisplayYMinimum=5.4248520785833119  ActiveDisplayYMaximum=17.175016435712966  DataLoggingVariableName=ScopeData5
  Subsystem1 : Subsystem
  Subsystem2 : Subsystem
  Sum3 : Sum  Inputs=|-+
  Sum4 : Sum  Inputs=|++
  Mass : Outport
  Ox Mass : Outport  Port=2
  Fuel Mass : Outport  Port=3
  wires:
  Thrust/1 -> Subsystem1/1(Thrust)
  Saturation1/1 -> Mass/1, Scope4/1
  Subsystem1/2(Ox_mdot) -> Subsystem2/1(Ox_mdot), Sum4/2
  Mass1/1 -> Sum3/2
  Integrator/1 -> Sum3/1
  Subsystem1/1(Fu_mdot) -> Sum4/1, Subsystem2/2(Fu_mdot)
  Sum3/1 -> Saturation1/1
  Sum4/1 -> Integrator/1
  Subsystem2/2(Fuel Mass) -> Fuel Mass/1, Scope13/1
  Subsystem2/1(Ox Mass) -> Ox Mass/1, Scope6/1

== system hopper_3dof_cascade_2/Subsystem2/If Action Subsystem ==
  In1 : Inport
  Action Port : ActionPort  ActionPortLabel=if(u1 < 0.2 & u2 < 0)
  Out1 : Outport
  wires:
  In1/1 -> Out1/1

== system hopper_3dof_cascade_2/Subsystem2/If Action Subsystem1 ==
  In1 : Inport
  Action Port : ActionPort  ActionPortLabel=else
  Gain : Gain  Gain=0
  Out1 : Outport
  wires:
  In1/1 -> Gain/1
  Gain/1 -> Out1/1

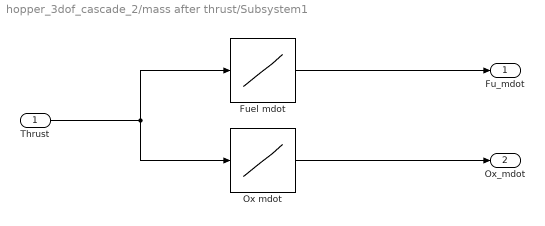
== system hopper_3dof_cascade_2/mass after thrust/Subsystem1 ==
  Thrust : Inport
  Fuel mdot : Lookup_n-D  NumberOfTableDimensions=1  BreakpointsForDimension1=bp  Table=tbl2  InternalRulePriority=Speed  RndMeth=Simplest
  Ox mdot : Lookup_n-D  NumberOfTableDimensions=1  BreakpointsForDimension1=bp  Table=tbl1  InternalRulePriority=Speed  RndMeth=Simplest
  Fu_mdot : Outport
  Ox_mdot : Outport  Port=2
  wires:
  Thrust/1 -> Ox mdot/1, Fuel mdot/1
  Fuel mdot/1 -> Fu_mdot/1
  Ox mdot/1 -> Ox_mdot/1

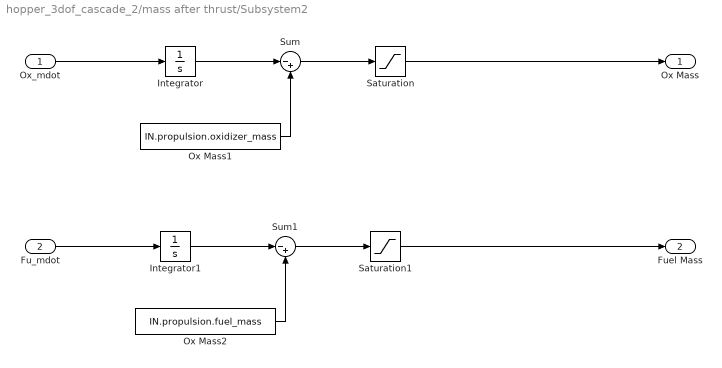
== system hopper_3dof_cascade_2/mass after thrust/Subsystem2 ==
  Ox_mdot : Inport
  Fu_mdot : Inport  Port=2
  Integrator : Integrator
  Integrator1 : Integrator
  Ox Mass1 : Constant  Value=IN.propulsion.oxidizer_mass
  Ox Mass2 : Constant  Value=IN.propulsion.fuel_mass
  Saturation : Saturate  UpperLimit=IN.propulsion.oxidizer_mass  LowerLimit=0
  Saturation1 : Saturate  UpperLimit=IN.propulsion.fuel_mass  LowerLimit=0
  Sum : Sum  Inputs=|-+
  Sum1 : Sum  Inputs=|-+
  Ox Mass : Outport
  Fuel Mass : Outport  Port=2
  wires:
  Ox_mdot/1 -> Integrator/1
  Integrator/1 -> Sum/1
  Ox Mass1/1 -> Sum/2
  Sum/1 -> Saturation/1
  Saturation/1 -> Ox Mass/1
  Sum1/1 -> Saturation1/1
  Saturation1/1 -> Fuel Mass/1
  Fu_mdot/1 -> Integrator1/1
  Ox Mass2/1 -> Sum1/2
  Integrator1/1 -> Sum1/1

== matlab function hopper_3dof_cascade_2/MATLAB Function ==
  data: t input; zref output
function zref = z_ref(t)
% Smooth realistic altitude trajectory

zf = 50;        % final altitude (m)
Tup = 14;       % ascent time (s)
Thover = 5;     % hover time (s)
Tdown = 20;     % descent time (s)

% Minimum-jerk profile
mjerk = @(s) (10*s.^3 - 15*s.^4 + 6*s.^5);

if t < 0
    zref = 0;

elseif t < Tup
    s = t / Tup;
    zref = zf * mjerk(s);

elseif t < Tup + Thover
    zref = zf;

elseif t < Tup + Thover + Tdown
    s = (t - (Tup + Thover)) / Tdown;
    zref = zf * (1 - mjerk(s));

else
    zref = 0;
end
